simulink model "test_codegen_sim_05"  (Simulink 7.9)
settings: Solver=VariableStepDiscrete  StartTime=0.0  StopTime=10.0  FixedStep=0.1  RelTol=1e-3
values from neighbouring files (symbols this model uses):
  model = mpt_import(sysStruct,probStruct)    [test_codegen_01_pass.m]    (also in test_codegen_02_pass.m; test_codegen_03_pass.m = LTISystem('A',dsys.A,'B',dsys.B,'C',dsys.C,'D',dsys.D, 'Ts',; test_codegen_04_pass.m = LTISystem('A',dsys.A,'B',dsys.B,'C',dsys.C,'D',dsys.D, 'Ts',; test_codegen_05_pass.m = PWASystem([mode1, mode2]))
  x0 = [X0; zeros(model.ny,1)]    [modelsim_sfunc.m]
undefined symbols (not defined in the file or in its folder): N
settings Model: Creator=mato  LastModifiedBy=mato
settings SolverCC: AutoInsertRateTranBlk=on

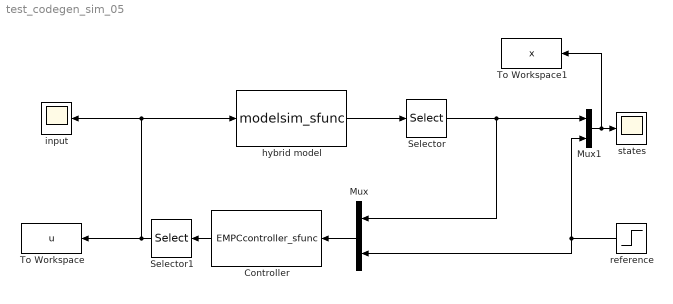
== system test_codegen_sim_05 ==
  Controller : S-Function  FunctionName=EMPCcontroller_sfunc  EnableBusSupport=off
  Mux : Mux  Inputs=2
  Mux1 : Mux  Inputs=2
  Selector : Selector  InputPortWidth=model.nx+model.ny  IndexOptions=Index vector (dialog)  Indices=1:model.nx  OutputSizes=1
  Selector1 : Selector  InputPortWidth=model.nu*N  IndexOptions=Index vector (dialog)  Indices=1  OutputSizes=1
  To Workspace : ToWorkspace  VariableName=u  SampleTime=0.1
  To Workspace1 : ToWorkspace  VariableName=x  SampleTime=0.1
  hybrid model : S-Function  FunctionName=modelsim_sfunc  Parameters=model,x0  EnableBusSupport=off
  input : Scope
      settings: SaveName=ScopeData2
  reference : Step  SampleTime=0
  states : Scope
      settings: TimeRange=10  SaveName=ScopeData3
  wires:
  Controller/1 -> Selector1/1
  Mux/1 -> Controller/1
  reference/1 -> Mux1/2, Mux/2
  Mux1/1 -> states/1, To Workspace1/1
  hybrid model/1 -> Selector/1
  Selector/1 -> Mux/1, Mux1/1
  Selector1/1 -> input/1, hybrid model/1, To Workspace/1
